simulink model "tb_pack_bms"  (R2026b)
model workspace (MAT data in the model file):
  TB.load_t = [0 10000000]
  TB.load_I = [0 0]
  TB.hv_t = [0 10000000]
  TB.hv_v = [0 0]
  TB.chg_t = [0 10000000]
  TB.chg_v = [0 0]
  TB.rst_t = [0 10000000]
  TB.rst_v = [0 0]
  TB.sd_t = [0 10000000]
  TB.sd_v = [0 0]
  TB.alive_freeze_t = 1000000000
  TB.dock_t = [0 10000000]
  TB.dock_v = [0 0]
  TB.shv_t = [0 10000000]
  TB.shv_v = [1 1]
  TB.sok_t = [0 10000000]
  TB.sok_v = [1 1]
  TB.T_amb = 298.15
  TB.G_solar = 0
  TB.chg_force = 0
  TB.chg_force_I = 100
  TB.flt_t = [0 10000000]
  TB.flt_v = [0 0]
  TB.fan_mode = 0
  TB.dec_fast = 1
  TB.dec_cmd = 1
  TB.V_gate = [30 35]
  TB.R_esr = 0.01
  TB.load_is_power = 0
  TB.stop_Vmin = 0
  TB.stop_SOCmin = -1
  TB.stop_SOCmax = 2
  TB.stop_on_done = 0
values from neighbouring files (symbols this model uses):
  P = local_temp(P, 318.15)    [pwr_case_def.m]    (also in pwr_case_run.m = C.pmod(P))
undefined symbols (not defined in the file or in its folder): Ts
libraries: simulink x15, nesl_utility x10, fl_lib x7, ee_lib x6, eeGeneralControl x4
settings Model: Creator=aomar  LastModifiedBy=aomar

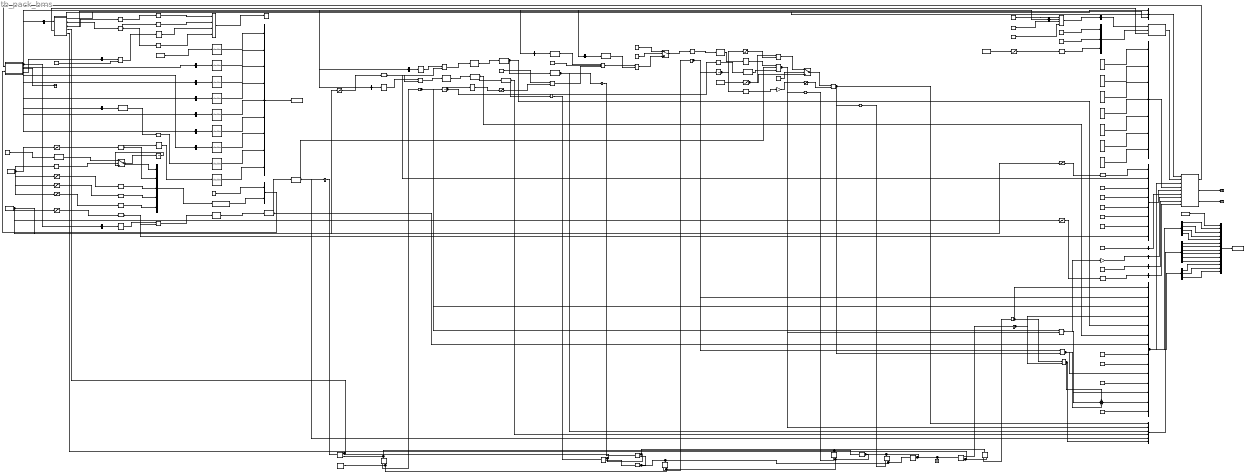
== system tb_pack_bms ==
  BMS : ModelReference  ModelNameDialog=Shaddad_BMS  SimulationMode=Normal  ModelReferenceVersion=1.1
  BMS_REQ_Pack : Subsystem  ReferencedSubsystem=bmsreq_can_pack
  Bal_log_sel : BusSelector  OutputSignals=Bal_Cmd
  Bal_sel : BusSelector  OutputSignals=Bal_Cmd
  Battery_Pack : Subsystem  Variant=on
  BmsReq_BC : BusCreator  Inputs=5  OutDataTypeStr=Bus: Bus_BmsReq  NonVirtualBus=on
      settings: InheritFromInputs=off
  C_bus : ee_lib/Passive/Capacitor  cap_option=ee.enum.passive.capacitor.capOption.const  c=P.power.pdu.C_bus_total_assumed F  Cvec=[1e-05, 1e-06] F  Vvec=[0, 10] V  CV_table_symmetry=ee.enum.passive.capacitor.tableSymmetry.yes  f_vec=[1, 10] kHz  DFext_vec=[.8, 1.2]  enable_C_tol=ee.enum.toleranceApplication.none  averaging_period=0 s  C_tol=5  tol_distribution=ee.enum.toleranceDistribution.uniform  nSigma=4  r=TB.R_esr Ohm  g=P.power.pdu.g_bleed 1/Ohm  enable_operating_limits=ee.enum.enable.no  operating_limit_action=ee.enum.passive.reportOpLim.warn  max_working_voltage_range=[-25, 25] V  power_rating=1 W  maxTemperature=85 degC  thermalEnable=false  thermalMass=1 J/K  i_specify=off  i_priority=None  i=0 A  i_nominal_specify=off  i_nominal_value=1  i_nominal_unit=A  v_specify=off  v_priority=None  v=0 V  v_nominal_specify=off  v_nominal_value=1  v_nominal_unit=V  vc_specify=on  vc_priority=High  vc=0 V  vc_nominal_specify=off  vc_nominal_value=1  vc_nominal_unit=V  T_specify=off  T_priority=None  T=298.15 K  T_nominal_specify=off  T_nominal_value=1  T_nominal_unit=K
  CanSlow_BC : BusCreator  Inputs=2  OutDataTypeStr=Bus: Bus_Can1_McuSlow  NonVirtualBus=on
      settings: InheritFromInputs=off
  Ch2_ok : Constant  Value=true  OutDataTypeStr=boolean  SampleTime=Ts.base
  Ch_ok : Constant  Value=true  OutDataTypeStr=boolean  SampleTime=Ts.base
  Charger : fl_lib/Electrical/Electrical Sources/Controlled Current Source
  Charger_BC : BusCreator  Inputs=1
  Charger_PS : nesl_utility/Simulink-PS Converter  PhysicalDomain=network_engine_domain  SubClassName=ps_input  LeftPortType=input  RightPortType=output  PseudoPeriodic=off  Frequencies=[]  NoiseDistribution=none  NoiseParameters=[]  Unit=A  AffineConversion=off  FilteringAndDerivatives=zero  SimscapeFilterOrder=1  InputFilterTimeConstant=0.001  UdotUserProvided=0
  Chg_RT : RateTransition  OutPortSampleTime=Ts.base
  Chg_en_dbl : DataTypeConversion  OutDataTypeStr=double  SaturateOnIntegerOverflow=off  RndMeth=Floor
  Chg_en_sel : BusSelector  OutputSignals=Charger_Enable
  Chg_force : Constant  Value=TB.chg_force  SampleTime=Ts.bms_fast
  Chg_force_I : Constant  Value=TB.chg_force_I  SampleTime=Ts.bms_fast
  Chg_force_sw : Switch  Criteria=u2 ~= 0  SaturateOnIntegerOverflow=off  InputSameDT=off
  Chg_lag : eeGeneralControl/Low-Pass Filter (Discrete or Continuous)  K=1  T=P.power.charger.tau  B=inf  A=-inf  init_option=Specify as parameter  x0=0  Ts=Ts.bms_fast
  Chg_slew : RateLimiter  RisingSlewLimit=P.power.charger.slew  FallingSlewLimit=-P.power.charger.slew  SampleTimeMode=inherited
  Clock_100ms : DigitalClock  SampleTime=Ts.env
  Clock_10ms : DigitalClock  SampleTime=Ts.bms_fast
  Clock_1ms : DigitalClock  SampleTime=Ts.base
  Clock_1ms_load : DigitalClock  SampleTime=Ts.base
  Clock_1ms_tab : DigitalClock  SampleTime=Ts.base
  Clock_50ms : DigitalClock  SampleTime=Ts.can_slow
  Dock_tab : Lookup_n-D  NumberOfTableDimensions=1  BreakpointsForDimension1=TB.dock_t  Table=TB.dock_v  InterpMethod=Flat  ExtrapMethod=Clip  InternalRulePriority=Speed  RndMeth=Simplest
  Dock_tab_100ms : Lookup_n-D  NumberOfTableDimensions=1  BreakpointsForDimension1=TB.dock_t  Table=TB.dock_v  InterpMethod=Flat  ExtrapMethod=Clip  InternalRulePriority=Speed  RndMeth=Simplest
  Dock_tab_100ms_b : simulink/Logic and Bit Operations/Compare To Zero  relop=~=  OutDataTypeStr=boolean
  Dock_tab_b : simulink/Logic and Bit Operations/Compare To Zero  relop=~=  OutDataTypeStr=boolean
  EStop_none : Constant  Value=false  OutDataTypeStr=boolean  SampleTime=Ts.base
  Env_BC : BusCreator  Inputs=3
  Env_ps_BC : BusCreator  Inputs=1
  Fan_BC : BusCreator  Inputs=1
  Fan_cmd_sel : BusSelector  OutputSignals=Fan_Cmd
  Fan_mode : Constant  Value=TB.fan_mode  SampleTime=Ts.bms_fast
  Fan_off : Constant  Value=single(0)  OutDataTypeStr=single  SampleTime=Ts.bms_fast
  Fan_on : Constant  Value=single(1)  OutDataTypeStr=single  SampleTime=Ts.bms_fast
  Fan_sel : MultiPortSwitch  DataPortOrder=Zero-based contiguous  zeroidx=on  SaturateOnIntegerOverflow=off  InputSameDT=off
  Fault_tab : Lookup_n-D  NumberOfTableDimensions=1  BreakpointsForDimension1=TB.flt_t  Table=TB.flt_v  InterpMethod=Flat  ExtrapMethod=Clip  InternalRulePriority=Speed  RndMeth=Simplest
  Fault_tab_b : simulink/Logic and Bit Operations/Compare To Zero  relop=~=  OutDataTypeStr=boolean
  Flt_BC : BusCreator  Inputs=1
  Fuse24_ok : Constant  Value=true  OutDataTypeStr=boolean  SampleTime=Ts.base
  FuseMain_ok : Constant  Value=true  OutDataTypeStr=boolean  SampleTime=Ts.base
  Fuse_ok : Constant  Value=true(6,1)  OutDataTypeStr=boolean  SampleTime=Ts.base
  GND : fl_lib/Electrical/Electrical Elements/Electrical Reference
  G_solar : Constant  Value=TB.G_solar  SampleTime=Ts.env
  HV_req_RT : RateTransition  OutPortSampleTime=Ts.bms_fast
  I_chg : Product  Inputs=3
  I_chg_en : Product
  I_chg_law : MinMax  Inputs=3
  I_chg_max : Constant  Value=P.power.charger.I_max  SampleTime=Ts.bms_fast
  I_from_P : Product  Inputs=*/
  I_load : Product
  I_pmax : Product  Inputs=*/
  I_req_dbl : DataTypeConversion  OutDataTypeStr=double  SaturateOnIntegerOverflow=off  RndMeth=Floor
  I_req_sel : BusSelector  OutputSignals=Charger_I_Req_A
  I_shunt : fl_lib/Electrical/Electrical Sensors/Current Sensor
  I_shunt_out : nesl_utility/PS-Simulink Converter  PhysicalDomain=network_engine_domain  SubClassName=ps_output  LeftPortType=input  RightPortType=output  PseudoPeriodic=off  Frequencies=[]  VectorFormat=inherit  Unit=inherit  AffineConversion=off
  Impl_BC : BusCreator  Inputs=1
  Impl_cmd_none : Constant  Value=P.ic.Bus_CanFrame8  OutDataTypeStr=Bus: Bus_CanFrame8  SampleTime=Ts.can_slow
  K1 : ee_lib/Switches & Breakers/Relays/SPST Relay  block_choices=ee.enum.controlport.ps  R_closed=P.power.pdu.K1.R_closed Ohm  G_open=P.power.pdu.K1.G_open 1/Ohm  Threshold=0.5  exposemeasurement=ee.enum.exposemeasurement.hidden  V_rated=5 V  V_energize=75  V_deenergize=25  l_winding=0.08 H  r_winding=12.5 Ohm  g_winding=1e-9 1/Ohm  T_brk_C_S=0 s  T_mak_C_S=0 s  fault_types=ee.enum.relays.faultTypes.winding
  K1_Cmd_sel : BusSelector  OutputSignals=K1_Cmd
  K1_aux : DataTypeConversion  OutDataTypeStr=boolean  SaturateOnIntegerOverflow=off  RndMeth=Floor
  K1_aux_dbl : DataTypeConversion  OutDataTypeStr=double  SaturateOnIntegerOverflow=off  RndMeth=Floor
  K1_cmd_RT : RateTransition  OutPortSampleTime=Ts.base
  K1_coil : Logic  AllPortsSameDT=off  OutDataTypeStr=boolean
  K1_coil_PS : nesl_utility/Simulink-PS Converter  PhysicalDomain=network_engine_domain  SubClassName=ps_input  LeftPortType=input  RightPortType=output  PseudoPeriodic=off  Frequencies=[]  NoiseDistribution=none  NoiseParameters=[]  Unit=1  AffineConversion=off  FilteringAndDerivatives=zero  SimscapeFilterOrder=1  InputFilterTimeConstant=0.001  UdotUserProvided=0
  K1_delay : eeGeneralControl/On-Off Delay  LabelModeActiveChoice=Discrete  Td_on=P.power.pdu.K1.t_on  Td_off=P.power.pdu.K1.t_off  IC=0  Ts=Ts.base
      settings: LibrarySourceBlock=ee_sl_lib/General Control/On-Off Delay
  K2 : ee_lib/Switches & Breakers/Relays/SPST Relay  block_choices=ee.enum.controlport.ps  R_closed=P.power.pdu.K2.R_closed Ohm  G_open=P.power.pdu.K2.G_open 1/Ohm  Threshold=0.5  exposemeasurement=ee.enum.exposemeasurement.hidden  V_rated=5 V  V_energize=75  V_deenergize=25  l_winding=0.08 H  r_winding=12.5 Ohm  g_winding=1e-9 1/Ohm  T_brk_C_S=0 s  T_mak_C_S=0 s  fault_types=ee.enum.relays.faultTypes.winding
  K2_Cmd_sel : BusSelector  OutputSignals=K2_Cmd
  K2_aux : DataTypeConversion  OutDataTypeStr=boolean  SaturateOnIntegerOverflow=off  RndMeth=Floor
  K2_aux_dbl : DataTypeConversion  OutDataTypeStr=double  SaturateOnIntegerOverflow=off  RndMeth=Floor
  K2_cmd_RT : RateTransition  OutPortSampleTime=Ts.base
  K2_coil : Logic  AllPortsSameDT=off  OutDataTypeStr=boolean
  K2_coil_PS : nesl_utility/Simulink-PS Converter  PhysicalDomain=network_engine_domain  SubClassName=ps_input  LeftPortType=input  RightPortType=output  PseudoPeriodic=off  Frequencies=[]  NoiseDistribution=none  NoiseParameters=[]  Unit=1  AffineConversion=off  FilteringAndDerivatives=zero  SimscapeFilterOrder=1  InputFilterTimeConstant=0.001  UdotUserProvided=0
  K2_delay : eeGeneralControl/On-Off Delay  LabelModeActiveChoice=Discrete  Td_on=P.power.pdu.K2.t_on  Td_off=P.power.pdu.K2.t_off  IC=0  Ts=Ts.base
      settings: LibrarySourceBlock=ee_sl_lib/General Control/On-Off Delay
  K3_none : Constant  Value=false  OutDataTypeStr=boolean  SampleTime=Ts.base
  K4 : ee_lib/Switches & Breakers/Relays/SPST Relay  block_choices=ee.enum.controlport.ps  R_closed=P.power.pdu.K4.R_closed Ohm  G_open=P.power.pdu.K4.G_open 1/Ohm  Threshold=0.5  exposemeasurement=ee.enum.exposemeasurement.hidden  V_rated=5 V  V_energize=75  V_deenergize=25  l_winding=0.08 H  r_winding=12.5 Ohm  g_winding=1e-9 1/Ohm  T_brk_C_S=0 s  T_mak_C_S=0 s  fault_types=ee.enum.relays.faultTypes.winding
  K4_Cmd_sel : BusSelector  OutputSignals=K4_Cmd
  K4_aux : DataTypeConversion  OutDataTypeStr=boolean  SaturateOnIntegerOverflow=off  RndMeth=Floor
  K4_aux_dbl : DataTypeConversion  OutDataTypeStr=double  SaturateOnIntegerOverflow=off  RndMeth=Floor
  K4_cmd_RT : RateTransition  OutPortSampleTime=Ts.base
  K4_coil : Logic  AllPortsSameDT=off  OutDataTypeStr=boolean
  K4_coil_PS : nesl_utility/Simulink-PS Converter  PhysicalDomain=network_engine_domain  SubClassName=ps_input  LeftPortType=input  RightPortType=output  PseudoPeriodic=off  Frequencies=[]  NoiseDistribution=none  NoiseParameters=[]  Unit=1  AffineConversion=off  FilteringAndDerivatives=zero  SimscapeFilterOrder=1  InputFilterTimeConstant=0.001  UdotUserProvided=0
  K4_delay : eeGeneralControl/On-Off Delay  LabelModeActiveChoice=Discrete  Td_on=P.power.pdu.K4.t_on  Td_off=P.power.pdu.K4.t_off  IC=0  Ts=Ts.base
      settings: LibrarySourceBlock=ee_sl_lib/General Control/On-Off Delay
  Key_on : Constant  Value=true  OutDataTypeStr=boolean  SampleTime=Ts.base
  Latched_none : Constant  Value=false  OutDataTypeStr=boolean  SampleTime=Ts.base
  Load : fl_lib/Electrical/Electrical Sources/Controlled Current Source
  Load_PS : nesl_utility/Simulink-PS Converter  PhysicalDomain=network_engine_domain  SubClassName=ps_input  LeftPortType=input  RightPortType=output  PseudoPeriodic=off  Frequencies=[]  NoiseDistribution=none  NoiseParameters=[]  Unit=A  AffineConversion=off  FilteringAndDerivatives=zero  SimscapeFilterOrder=1  InputFilterTimeConstant=0.001  UdotUserProvided=0
  Load_is_power : Constant  Value=TB.load_is_power  SampleTime=Ts.base
  Load_mode : Switch  Criteria=u2 ~= 0  SaturateOnIntegerOverflow=off  InputSameDT=off
  Load_tab : Lookup_n-D  NumberOfTableDimensions=1  BreakpointsForDimension1=TB.load_t  Table=TB.load_I  InterpMethod=Flat  ExtrapMethod=Clip  InternalRulePriority=Speed  RndMeth=Simplest
  Log_Charger_Enable_sel : BusSelector  OutputSignals=Charger_Enable
  Log_Charger_I_Req_A_sel : BusSelector  OutputSignals=Charger_I_Req_A
  Log_Fan_Cmd_sel : BusSelector  OutputSignals=Fan_Cmd
  Log_K1_Cmd_sel : BusSelector  OutputSignals=K1_Cmd
  Log_K2_Cmd_sel : BusSelector  OutputSignals=K2_Cmd
  Log_K4_Cmd_sel : BusSelector  OutputSignals=K4_Cmd
  Log_meas_sel : BusSelector  OutputSignals=V_pack,V_bus,V_dock,I_pack
  Log_pwr_sel : BusSelector  OutputSignals=P_trac_L,P_chg_bus,P_pdu_loss
  Log_stub_BC : BusCreator  Inputs=6
  Log_stub_sel : BusSelector  OutputSignals=I_load,I_chg,K1_closed_dbl,K2_closed_dbl,K4_closed_dbl,P_pack
  Lv_BC : BusCreator  Inputs=7
  MCU_Charge_Enable_Req : Lookup_n-D  NumberOfTableDimensions=1  BreakpointsForDimension1=TB.chg_t  Table=TB.chg_v  InterpMethod=Flat  ExtrapMethod=Clip  InternalRulePriority=Speed  RndMeth=Simplest
  MCU_Charge_Enable_Req_b : simulink/Logic and Bit Operations/Compare To Zero  relop=~=  OutDataTypeStr=boolean
  MCU_Fault_Reset_Req : Lookup_n-D  NumberOfTableDimensions=1  BreakpointsForDimension1=TB.rst_t  Table=TB.rst_v  InterpMethod=Flat  ExtrapMethod=Clip  InternalRulePriority=Speed  RndMeth=Simplest
  MCU_Fault_Reset_Req_b : simulink/Logic and Bit Operations/Compare To Zero  relop=~=  OutDataTypeStr=boolean
  MCU_HV_Enable_Req : Lookup_n-D  NumberOfTableDimensions=1  BreakpointsForDimension1=TB.hv_t  Table=TB.hv_v  InterpMethod=Flat  ExtrapMethod=Clip  InternalRulePriority=Speed  RndMeth=Simplest
  MCU_HV_Enable_Req_b : simulink/Logic and Bit Operations/Compare To Zero  relop=~=  OutDataTypeStr=boolean
  MCU_Shutdown_Req : Lookup_n-D  NumberOfTableDimensions=1  BreakpointsForDimension1=TB.sd_t  Table=TB.sd_v  InterpMethod=Flat  ExtrapMethod=Clip  InternalRulePriority=Speed  RndMeth=Simplest
  MCU_Shutdown_Req_b : simulink/Logic and Bit Operations/Compare To Zero  relop=~=  OutDataTypeStr=boolean
  MCU_alive : simulink/Sources/Counter Free-Running  NumBits=8  tsamp=Ts.can_slow
  MCU_alive_hold : UnitDelay  InitialCondition=uint8(0)  SampleTime=Ts.can_slow
  MCU_alive_run : simulink/Logic and Bit Operations/Compare To Constant  relop=<  const=TB.alive_freeze_t  OutDataTypeStr=boolean
  MCU_alive_sw : Switch  Criteria=u2 ~= 0  SaturateOnIntegerOverflow=off  InputSameDT=off
  MCU_alive_u8 : DataTypeConversion  OutDataTypeStr=uint8  SaturateOnIntegerOverflow=off  RndMeth=Floor
  OVP_ok : simulink/Logic and Bit Operations/Compare To Constant  relop=<  const=P.power.charger.V_ovp  OutDataTypeStr=boolean
  OVP_ok_dbl : DataTypeConversion  OutDataTypeStr=double  SaturateOnIntegerOverflow=off  RndMeth=Floor
  P_chg_bus : Product
  P_chg_max : Constant  Value=P.power.charger.P_max  SampleTime=Ts.bms_fast
  P_grid : Gain  Gain=1/P.power.charger.eta
  P_pack : Product
  P_pdu_loss : Sum  Inputs=++-
  P_trac : Product
  Pack_BC : BusCreator  Inputs=3
  Pack_Thermal : Subsystem  ReferencedSubsystem=Pack_Thermal
  Pdu_BC : BusCreator  Inputs=14
  Power_Sensors : Subsystem  ReferencedSubsystem=Power_Sensors
  R_dock_bleed : ee_lib/Passive/Resistor  R=P.power.charger.R_bleed Ohm  enable_R_tol=ee.enum.toleranceApplication.none  R_tol=5  tol_distribution=ee.enum.toleranceDistribution.uniform  nSigma=4  enable_operating_limits=ee.enum.enable.no  operating_limit_action=ee.enum.passive.reportOpLim.warn  power_rating=1 W  max_working_voltage=100 V  noise_mode=ee.enum.sources.noise.Disabled  Tdevice=25 degC  sample_time=1e-3 s  repeatability=ee.enum.ic.repeatability.notRepeatable  user_seed=0  auto_seed=2562091618  power_derating_T1=70 degC  power_derating_T2=155 degC  operating_temperature_range_vec=[-50, 150] degC  alpha=3.93e-3 1/K  Tmeas=25 degC  thermal_mass=100 J/K  temperature_specify=off  temperature_priority=High  temperature=298.15 K  temperature_nominal_specify=off  temperature_nominal_value=1  temperature_nominal_unit=K
  R_pre : ee_lib/Passive/Resistor  R=P.power.pdu.R_pre Ohm  enable_R_tol=ee.enum.toleranceApplication.none  R_tol=5  tol_distribution=ee.enum.toleranceDistribution.uniform  nSigma=4  enable_operating_limits=ee.enum.enable.no  operating_limit_action=ee.enum.passive.reportOpLim.warn  power_rating=1 W  max_working_voltage=100 V  noise_mode=ee.enum.sources.noise.Disabled  Tdevice=25 degC  sample_time=1e-3 s  repeatability=ee.enum.ic.repeatability.notRepeatable  user_seed=0  auto_seed=4166091829  power_derating_T1=70 degC  power_derating_T2=155 degC  operating_temperature_range_vec=[-50, 150] degC  alpha=3.93e-3 1/K  Tmeas=25 degC  thermal_mass=100 J/K  temperature_specify=off  temperature_priority=High  temperature=298.15 K  temperature_nominal_specify=off  temperature_nominal_value=1  temperature_nominal_unit=K
  Rails : Constant  Value=[24; 2; 24; 12; 4; 5; 3.3]  SampleTime=Ts.base
  Rails_ok : Constant  Value=true(4,1)  OutDataTypeStr=boolean  SampleTime=Ts.base
  SOC_min_true : MinMax
  Safety_BC : BusCreator  Inputs=8
  Safety_HV_OK_tab : Lookup_n-D  NumberOfTableDimensions=1  BreakpointsForDimension1=TB.shv_t  Table=TB.shv_v  InterpMethod=Flat  ExtrapMethod=Clip  InternalRulePriority=Speed  RndMeth=Simplest
  Safety_HV_OK_tab_b : simulink/Logic and Bit Operations/Compare To Zero  relop=~=  OutDataTypeStr=boolean
  Safety_OK_tab : Lookup_n-D  NumberOfTableDimensions=1  BreakpointsForDimension1=TB.sok_t  Table=TB.sok_v  InterpMethod=Flat  ExtrapMethod=Clip  InternalRulePriority=Speed  RndMeth=Simplest
  Safety_OK_tab_b : simulink/Logic and Bit Operations/Compare To Zero  relop=~=  OutDataTypeStr=boolean
  Solver : nesl_utility/Solver Configuration  PhysicalDomain=network_engine_domain  SubClassName=solver  LeftPortType=input  RightPortType=generic  Tones=[]  Harmonics=[]  SimulateNoise=off  Profile=off  UseLocalSampling=off  EnableSwitchedLinearOptims=on  FrequencyDomain=off  UseCCode=off  RelTol=0.001  AbsTol=0.001  MinStep=1e-09  ToWorkspace=off  RevertToSquareIcSolve=off  NumHomotopyIterations=100  PhasorMode=off  PhasorModeNumHarmonics=1  ConsistencySolver=NEWTON_XTOL_AFTER_FTOL  CanonicalOrdering=CANONICAL  OptimizeIntermediates=OPTIMIZED  MulticoreSolverChoice=BACKWARD_EULER  IndexReductionMethod=DerivativeReplacement  DoDC=off  ResidualTolerance=1e-09  ConsistencyTolSource=GLOBAL  ConsistencyAbsTol=0.001  ConsistencyRelTol=0.001  ConsistencyTolFactor=0.001  UseLocalSolver=on  LocalSolverChoice=NE_BACKWARD_EULER_ADVANCER  ResolveIndetEquations=on  FunctionEvalNumThread=1  LocalSolverSampleTime=P.sim.ssc.Ts  DoFixedCost=on  MaxNonlinIter=P.power.tb.MaxNonlinIter  MaxModeIter=P.power.tb.MaxModeIter  ComputeImpulses=off  ImpulseIterations=2  LinearAlgebra=auto  LinearAlgebraNumThread=0  EquationFormulation=NE_TIME_EF  DelaysMemoryBudget=1024  AutomaticFiltering=on  FilteringTimeConstant=0.001  PartitionStorageMethod=AS_NEEDED  PartitionMemoryBudget=1024  PartitionMethod=BALANCED  MultibodyUseLocalSolver=off  MultibodyLocalSolverChoice=ODE1  MultibodyLocalSolverSampleTime=0.001
  Stop : Stop
  Stop_SOC : simulink/Logic and Bit Operations/Compare To Constant  relop=<  const=TB.stop_SOCmin  OutDataTypeStr=boolean
  Stop_SOCmax : simulink/Logic and Bit Operations/Compare To Constant  relop=>  const=TB.stop_SOCmax  OutDataTypeStr=boolean
  Stop_V : simulink/Logic and Bit Operations/Compare To Constant  relop=<  const=TB.stop_Vmin  OutDataTypeStr=boolean
  Stop_any : Logic  Operator=OR  Inputs=4  AllPortsSameDT=off  OutDataTypeStr=boolean
  Stop_done : Logic  AllPortsSameDT=off  OutDataTypeStr=boolean
  Stop_done_RT : RateTransition  OutPortSampleTime=Ts.base
  Stop_on_done : Constant  Value=TB.stop_on_done  OutDataTypeStr=boolean  SampleTime=Ts.hk
  T_amb : Constant  Value=TB.T_amb  SampleTime=Ts.env
  T_amb_ps : Constant  Value=TB.T_amb  SampleTime=Ts.env
  Telem_sel : BusSelector  OutputSignals=Charge_Complete
  V_bus_d : UnitDelay  SampleTime=Ts.base
  V_bus_min : Saturate  UpperLimit=inf  LowerLimit=30
  V_bus_sens : fl_lib/Electrical/Electrical Sensors/Voltage Sensor
  V_bus_sens_out : nesl_utility/PS-Simulink Converter  PhysicalDomain=network_engine_domain  SubClassName=ps_output  LeftPortType=input  RightPortType=output  PseudoPeriodic=off  Frequencies=[]  VectorFormat=inherit  Unit=inherit  AffineConversion=off
  V_dock_RT : RateTransition  OutPortSampleTime=Ts.bms_fast
  V_dock_d : UnitDelay  SampleTime=Ts.base
  V_dock_min : Saturate  UpperLimit=inf  LowerLimit=1
  V_dock_sens : fl_lib/Electrical/Electrical Sensors/Voltage Sensor
  V_dock_sens_out : nesl_utility/PS-Simulink Converter  PhysicalDomain=network_engine_domain  SubClassName=ps_output  LeftPortType=input  RightPortType=output  PseudoPeriodic=off  Frequencies=[]  VectorFormat=inherit  Unit=inherit  AffineConversion=off
  V_gate : Saturate  UpperLimit=1  LowerLimit=0
  V_gate_k : Gain  Gain=1/(TB.V_gate(2) - TB.V_gate(1))
  V_gate_off : Bias  Bias=-TB.V_gate(1)  SaturateOnIntegerOverflow=off
  V_pack_sens : fl_lib/Electrical/Electrical Sensors/Voltage Sensor
  V_pack_sens_out : nesl_utility/PS-Simulink Converter  PhysicalDomain=network_engine_domain  SubClassName=ps_output  LeftPortType=input  RightPortType=output  PseudoPeriodic=off  Frequencies=[]  VectorFormat=inherit  Unit=inherit  AffineConversion=off
  Vcell_min_true : MinMax
  Zero_P_bms : Constant  Value=0  SampleTime=Ts.base
  Zero_P_dcdc_loss : Constant  Value=0  SampleTime=Ts.base
  Zero_P_impl : Constant  Value=0  SampleTime=Ts.base
  Zero_P_k3_loss : Constant  Value=0  SampleTime=Ts.base
  Zero_P_lv : Constant  Value=0  SampleTime=Ts.base
  Zero_P_trac_R : Constant  Value=0  SampleTime=Ts.base
  can_tx_term : Terminator
  lc_dbl{1..9} (9 alike) : DataTypeConversion  OutDataTypeStr=double  SaturateOnIntegerOverflow=off  RndMeth=Floor
  log_cmd : ToWorkspace  VariableName=log_cmd  SampleTime=-1
      settings: Decimation=TB.dec_cmd
  log_cmd_mux : Mux  Inputs=9
  log_fast : ToWorkspace  VariableName=log_fast  SampleTime=-1
      settings: Decimation=TB.dec_fast
  log_fast_mux : Mux  Inputs=14
  n_bal_dbl : DataTypeConversion  OutDataTypeStr=double  SaturateOnIntegerOverflow=off  RndMeth=Floor
  n_bal_sum : Sum  Inputs=+
  status_term : Terminator
  truth_term : Terminator
  wires:
  MCU_alive/1 -> MCU_alive_u8/1  "alive_count"
  Clock_1ms_tab/1 -> Safety_HV_OK_tab/1, Safety_OK_tab/1, Fault_tab/1, Dock_tab/1  "t_1ms_tab"
  Clock_50ms/1 -> MCU_HV_Enable_Req/1, MCU_Shutdown_Req/1, MCU_Fault_Reset_Req/1, MCU_alive_run/1, MCU_Charge_Enable_Req/1  "t_50ms"
  BMS/1 -> K4_Cmd_sel/1, Log_Fan_Cmd_sel/1, Log_Charger_I_Req_A_sel/1, Log_Charger_Enable_sel/1, Fan_cmd_sel/1, Bal_sel/1, Bal_log_sel/1, Log_K4_Cmd_sel/1, K2_Cmd_sel/1, Log_K2_Cmd_sel/1, I_req_sel/1, Chg_en_sel/1, K1_Cmd_sel/1, Log_K1_Cmd_sel/1  "bms_cmd"
  BMS/2 -> can_tx_term/1  "can_tx"
  BMS/3 -> Telem_sel/1  "telem"
  Bal_sel/1 -> Battery_Pack/1(Bal_Cmd)  "<Bal_Cmd>"
  Stop_on_done/1 -> Stop_done/2  "stop_on_done"
  MCU_alive_run/1 -> MCU_alive_sw/2  "alive_running"
  MCU_HV_Enable_Req/1 -> MCU_HV_Enable_Req_b/1  "HV_Enable_Req_tab"
  MCU_Charge_Enable_Req/1 -> MCU_Charge_Enable_Req_b/1  "Charge_Enable_Req_tab"
  MCU_Fault_Reset_Req/1 -> MCU_Fault_Reset_Req_b/1  "Fault_Reset_Req_tab"
  MCU_Shutdown_Req/1 -> MCU_Shutdown_Req_b/1  "Shutdown_Req_tab"
  Dock_tab/1 -> Dock_tab_b/1  "dock_present_tab"
  MCU_alive_u8/1 -> MCU_alive_sw/1  "alive_count_u8"
  Battery_Pack/1(T_cell_true) -> Pack_BC/1  "T_cell_true"
  Telem_sel/1 -> Stop_done/1  "<Charge_Complete>"
  Bal_log_sel/1 -> n_bal_dbl/1  "<Bal_Cmd>"
  K4_Cmd_sel/1 -> K4_cmd_RT/1  "<K4_Cmd>"
  Vcell_min_true/1 -> Stop_V/1  "V_cell_min"
  SOC_min_true/1 -> Stop_SOCmax/1, Stop_SOC/1  "SOC_min"
  Stop_done/1 -> Stop_done_RT/1  "stop_done"
  MCU_HV_Enable_Req_b/1 -> BmsReq_BC/2, HV_req_RT/1  "HV_Enable_Req"
  MCU_Charge_Enable_Req_b/1 -> BmsReq_BC/3  "Charge_Enable_Req"
  MCU_Fault_Reset_Req_b/1 -> BmsReq_BC/4  "Fault_Reset_Req"
  MCU_Shutdown_Req_b/1 -> BmsReq_BC/5  "Shutdown_Req"
  Dock_tab_b/1 -> Safety_BC/8, K4_coil/2  "dock_present"
  K4_cmd_RT/1 -> K4_coil/1  "K4_Cmd_1ms"
  MCU_alive_sw/1 -> MCU_alive_hold/1, BmsReq_BC/1  "AliveCounter"
  n_bal_dbl/1 -> n_bal_sum/1  "Bal_Cmd_dbl"
  BmsReq_BC/1 -> BMS_REQ_Pack/1  "bms_req"
  Stop_V/1 -> Stop_any/1  "stop_V"
  Stop_SOC/1 -> Stop_any/2  "stop_SOC"
  Stop_SOCmax/1 -> Stop_any/4  "stop_SOCmax"
  n_bal_sum/1 -> lc_dbl8/1  "n_Bal"
  K4_coil/1 -> K4_delay/1  "K4_coil"
  MCU_alive_hold/1 -> MCU_alive_sw/3  "alive_held"
  Stop_done_RT/1 -> Stop_any/3  "stop_done_1ms"
  HV_req_RT/1 -> lc_dbl9/1  "HV_Enable_Req_10ms"
  Clock_10ms/1 -> lc_dbl1/1  "t_10ms"
  Log_K1_Cmd_sel/1 -> lc_dbl2/1  "<K1_Cmd>"
  Log_K2_Cmd_sel/1 -> lc_dbl3/1  "<K2_Cmd>"
  Log_K4_Cmd_sel/1 -> lc_dbl4/1  "<K4_Cmd>"
  Log_Charger_Enable_sel/1 -> lc_dbl5/1  "<Charger_Enable>"
  Log_Charger_I_Req_A_sel/1 -> lc_dbl6/1  "<Charger_I_Req_A>"
  Log_Fan_Cmd_sel/1 -> lc_dbl7/1  "<Fan_Cmd>"
  Stop_any/1 -> Stop/1  "stop_run"
  Impl_cmd_none/1 -> CanSlow_BC/1  "impl_cmd"
  K4_delay/1 -> K4_aux/1  "K4_contact"
  lc_dbl1/1 -> log_cmd_mux/1  "t_dbl"
  lc_dbl2/1 -> log_cmd_mux/2  "K1_Cmd_dbl"
  lc_dbl3/1 -> log_cmd_mux/3  "K2_Cmd_dbl"
  lc_dbl4/1 -> log_cmd_mux/4  "K4_Cmd_dbl"
  lc_dbl5/1 -> log_cmd_mux/5  "Charger_Enable_dbl"
  lc_dbl6/1 -> log_cmd_mux/6  "I_req_dbl"
  lc_dbl7/1 -> log_cmd_mux/7  "Fan_Cmd_dbl"
  lc_dbl8/1 -> log_cmd_mux/8  "n_Bal_dbl"
  lc_dbl9/1 -> log_cmd_mux/9  "HV_Enable_Req_MCU_dbl"
  BMS_REQ_Pack/1 -> CanSlow_BC/2  "bms_req"
  log_cmd_mux/1 -> log_cmd/1  "log_cmd"
  CanSlow_BC/1 -> BMS/2  "can_rx"
  K4_aux/1 -> Pdu_BC/7, K4_aux_dbl/1  "K4_closed"
  K4_aux_dbl/1 -> Log_stub_BC/5, I_chg/2, K4_coil_PS/1  "K4_closed_dbl"
  Safety_HV_OK_tab/1 -> Safety_HV_OK_tab_b/1  "Safety_HV_OK_tab"
  K2_Cmd_sel/1 -> K2_cmd_RT/1  "<K2_Cmd>"
  Safety_HV_OK_tab_b/1 -> Safety_BC/2, K2_coil/2, K1_coil/2  "Safety_HV_OK"
  K2_cmd_RT/1 -> K2_coil/1  "K2_Cmd_1ms"
  K1_Cmd_sel/1 -> K1_cmd_RT/1  "<K1_Cmd>"
  V_dock_sens_out/1 -> P_chg_bus/1, Pdu_BC/3, V_dock_d/1  "V_dock"
  K2_coil/1 -> K2_delay/1  "K2_coil"
  K1_cmd_RT/1 -> K1_coil/1  "K1_Cmd_1ms"
  K1_coil/1 -> K1_delay/1  "K1_coil"
  V_dock_d/1 -> OVP_ok/1, V_dock_RT/1  "V_dock_d"
  K2_delay/1 -> K2_aux/1  "K2_contact"
  V_dock_RT/1 -> V_dock_min/1  "V_dock_10ms"
  K1_delay/1 -> K1_aux/1  "K1_contact"
  K2_aux/1 -> Pdu_BC/6, K2_aux_dbl/1  "K2_closed"
  P_chg_max/1 -> I_pmax/1  "P_chg_max"
  V_dock_min/1 -> I_pmax/2  "V_dock_min"
  K1_aux/1 -> Pdu_BC/5, K1_aux_dbl/1  "K1_closed"
  K2_aux_dbl/1 -> Log_stub_BC/4, K2_coil_PS/1  "K2_closed_dbl"
  I_req_sel/1 -> I_req_dbl/1  "<Charger_I_Req_A>"
  I_chg_max/1 -> I_chg_law/2  "I_chg_max"
  I_pmax/1 -> I_chg_law/3  "I_pmax"
  I_req_dbl/1 -> I_chg_law/1  "I_req"
  K1_aux_dbl/1 -> Log_stub_BC/3, K1_coil_PS/1  "K1_closed_dbl"
  Chg_en_sel/1 -> Chg_en_dbl/1  "<Charger_Enable>"
  I_chg_law/1 -> I_chg_en/1  "I_chg_law"
  Chg_en_dbl/1 -> I_chg_en/2  "charger_enable"
  Chg_force_I/1 -> Chg_force_sw/1  "chg_force_I"
  Chg_force/1 -> Chg_force_sw/2  "chg_force"
  I_chg_en/1 -> Chg_force_sw/3  "I_chg_cmd"
  Chg_force_sw/1 -> Chg_slew/1  "I_chg_target"
  V_bus_sens_out/1 -> P_trac/1, Pdu_BC/2, V_bus_d/1  "V_bus"
  Chg_slew/1 -> Chg_lag/1  "I_chg_slewed"
  OVP_ok/1 -> OVP_ok_dbl/1  "ovp_ok"
  V_bus_d/1 -> V_bus_min/1, V_gate_off/1  "V_bus_d"
  Clock_1ms_load/1 -> Load_tab/1  "t_1ms_load"
  Chg_lag/1 -> Chg_RT/1  "I_chg_set"
  V_bus_min/1 -> I_from_P/2  "V_bus_d_min"
  Chg_RT/1 -> I_chg/1  "I_chg_set_1ms"
  Load_tab/1 -> I_from_P/1, Load_mode/3  "load_tab"
  V_gate_off/1 -> V_gate_k/1  "V_gate_dV"
  OVP_ok_dbl/1 -> I_chg/3  "ovp_ok_dbl"
  I_from_P/1 -> Load_mode/1  "I_from_P"
  I_chg/1 -> Log_stub_BC/2, P_chg_bus/2, Charger_PS/1  "I_chg"
  Load_is_power/1 -> Load_mode/2  "load_is_power"
  V_gate_k/1 -> V_gate/1  "V_gate_raw"
  V_gate/1 -> I_load/2  "V_gate"
  Load_mode/1 -> I_load/1  "I_load_req"
  I_load/1 -> Log_stub_BC/1, P_trac/2, Load_PS/1  "I_load"
  Clock_100ms/1 -> Dock_tab_100ms/1  "t_100ms"
  V_pack_sens_out/1 -> P_pack/1, Pdu_BC/1  "V_pack"
  I_shunt_out/1 -> P_pack/2, Pdu_BC/4  "I_pack"
  Fan_mode/1 -> Fan_sel/1  "fan_mode"
  Fan_off/1 -> Fan_sel/3  "fan_off"
  Fan_on/1 -> Fan_sel/4  "fan_on"
  Dock_tab_100ms/1 -> Dock_tab_100ms_b/1  "dock_contact_tab"
  Fan_cmd_sel/1 -> Fan_sel/2  "<Fan_Cmd>"
  T_amb/1 -> Env_BC/1  "T_amb"
  G_solar/1 -> Env_BC/2  "G_solar"
  P_chg_bus/1 -> P_grid/1, P_pdu_loss/2, Pdu_BC/12  "P_chg_bus"
  Fan_sel/1 -> Fan_BC/1  "Fan_Cmd"
  Dock_tab_100ms_b/1 -> Env_BC/3  "dock_contact"
  Safety_OK_tab/1 -> Safety_OK_tab_b/1  "Safety_OK_tab"
  Fault_tab/1 -> Fault_tab_b/1  "bms_fault_tab"
  P_trac/1 -> P_pdu_loss/3, Pdu_BC/10  "P_trac_L"
  P_pack/1 -> Log_stub_BC/6, P_pdu_loss/1  "P_pack"
  Fan_BC/1 -> Pack_Thermal/1  "fan_cmd"
  Env_BC/1 -> Pack_Thermal/2  "env"
  P_pdu_loss/1 -> Pdu_BC/13  "P_pdu_loss"
  Rails/1 -> Lv_BC/1  "rails"
  Rails_ok/1 -> Lv_BC/2  "rail_ok"
  K3_none/1 -> Lv_BC/3  "K3_closed"
  Fuse24_ok/1 -> Lv_BC/4  "fuse24_ok"
  Zero_P_lv/1 -> Lv_BC/5  "P_lv"
  Zero_P_dcdc_loss/1 -> Lv_BC/6  "P_dcdc_loss"
  Zero_P_k3_loss/1 -> Lv_BC/7  "P_k3_loss"
  EStop_none/1 -> Safety_BC/3  "EStop_Any"
  Ch_ok/1 -> Safety_BC/4  "EStop_Ch1_OK"
  Ch2_ok/1 -> Safety_BC/5  "EStop_Ch2_OK"
  Latched_none/1 -> Safety_BC/6  "Safety_Latched_Off"
  Key_on/1 -> Safety_BC/7  "key_on"
  Zero_P_impl/1 -> Impl_BC/1  "P_impl"
  P_grid/1 -> Charger_BC/1  "P_grid"
  T_amb_ps/1 -> Env_ps_BC/1  "T_amb"
  Fuse_ok/1 -> Pdu_BC/8  "fuse_ok"
  FuseMain_ok/1 -> Pdu_BC/9  "F_MAIN_ok"
  Zero_P_trac_R/1 -> Pdu_BC/11  "P_trac_R"
  Zero_P_bms/1 -> Pdu_BC/14  "P_bms"
  Safety_OK_tab_b/1 -> Safety_BC/1  "Safety_OK"
  Fault_tab_b/1 -> Flt_BC/1  "bms_fault"
  Pack_BC/1 -> Power_Sensors/1  "pack"
  Lv_BC/1 -> Power_Sensors/4  "lv"
  Safety_BC/1 -> Power_Sensors/5  "safety"
  Impl_BC/1 -> Power_Sensors/6  "impl"
  Charger_BC/1 -> Power_Sensors/7  "charger"
  Env_ps_BC/1 -> Power_Sensors/8  "env"
  Flt_BC/1 -> Power_Sensors/9  "flt"
  Pdu_BC/1 -> Power_Sensors/3, Log_meas_sel/1, Log_pwr_sel/1  "pdu"
  Log_stub_BC/1 -> Log_stub_sel/1  "log_stub"
  Pack_Thermal/1 -> Power_Sensors/2  "thermal"
  Log_meas_sel/1 -> log_fast_mux/2  "<V_pack>"
  Log_meas_sel/2 -> log_fast_mux/3  "<V_bus>"
  Log_meas_sel/3 -> log_fast_mux/4  "<V_dock>"
  Log_meas_sel/4 -> log_fast_mux/5  "<I_pack>"
  Log_stub_sel/1 -> log_fast_mux/6  "<I_load>"
  Log_stub_sel/2 -> log_fast_mux/7  "<I_chg>"
  Log_stub_sel/3 -> log_fast_mux/8  "<K1_closed_dbl>"
  Log_stub_sel/4 -> log_fast_mux/9  "<K2_closed_dbl>"
  Log_stub_sel/5 -> log_fast_mux/10  "<K4_closed_dbl>"
  Log_stub_sel/6 -> log_fast_mux/11  "<P_pack>"
  Log_pwr_sel/1 -> log_fast_mux/12  "<P_trac_L>"
  Log_pwr_sel/2 -> log_fast_mux/13  "<P_chg_bus>"
  Log_pwr_sel/3 -> log_fast_mux/14  "<P_pdu_loss>"
  Clock_1ms/1 -> log_fast_mux/1  "t_1ms"
  Power_Sensors/1 -> BMS/1  "bms_meas"
  Power_Sensors/2 -> status_term/1  "power_status"
  Power_Sensors/3 -> truth_term/1  "power_truth"
  log_fast_mux/1 -> log_fast/1  "log_fast"
  Battery_Pack/2(SOC_true) -> SOC_min_true/1, Pack_BC/2  "SOC_true"
  Battery_Pack/3(V_cell_true) -> Pack_BC/3, Vcell_min_true/1  "V_cell_true"
  connections:
  Battery_Pack/LConn1 -- Pack_Thermal/LConn1
  K4/RConn1 -- Battery_Pack/RConn1 -- K2/RConn1 -- K1/RConn1 -- V_pack_sens/LConn1
  I_shunt/RConn2 -- Battery_Pack/RConn2 -- V_pack_sens/RConn2
  R_pre/RConn1 -- K1/RConn2 -- V_bus_sens/LConn1 -- Load/RConn2 -- C_bus/LConn1
  V_dock_sens/RConn2 -- Solver/RConn1 -- V_bus_sens/RConn2 -- Charger/RConn2 -- R_dock_bleed/RConn1 -- Load/LConn1 -- C_bus/RConn1 -- GND/LConn1 -- I_shunt/LConn1
  V_dock_sens/LConn1 -- K4/RConn2 -- Charger/LConn1 -- R_dock_bleed/LConn1
  Charger_PS/RConn1 -- Charger/RConn1
  I_shunt_out/LConn1 -- I_shunt/RConn1
  K1_coil_PS/RConn1 -- K1/LConn1
  K2_coil_PS/RConn1 -- K2/LConn1
  K2/RConn2 -- R_pre/LConn1
  K4_coil_PS/RConn1 -- K4/LConn1
  Load_PS/RConn1 -- Load/RConn1
  V_bus_sens_out/LConn1 -- V_bus_sens/RConn1
  V_dock_sens_out/LConn1 -- V_dock_sens/RConn1
  V_pack_sens_out/LConn1 -- V_pack_sens/RConn1

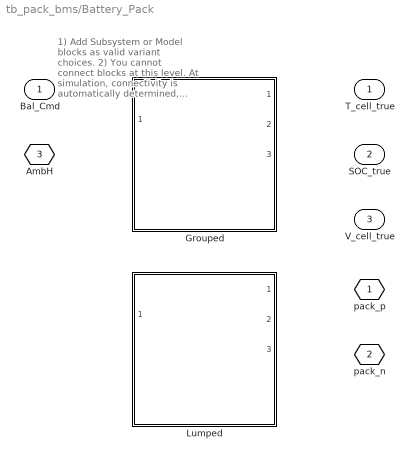
== system tb_pack_bms/Battery_Pack ==
  note: 1) Add Subsystem or Model blocks as valid variant choices.
      | 2) You cannot connect blocks at this level. At simulation, connectivity is automatically
      | determined, based on the active variant and port name matching.
  Bal_Cmd : Inport
  Grouped : Subsystem  VariantControl=VC_PACK == 1  ReferencedSubsystem=Pack_Grouped
  Lumped : Subsystem  VariantControl=VC_PACK == 2  ReferencedSubsystem=Pack_Lumped
  pack_p : PMIOPort  Side=Right  ConnectionType=Connection: foundation.electrical.electrical
  pack_n : PMIOPort  Port=2  Side=Right  ConnectionType=Connection: foundation.electrical.electrical
  AmbH : PMIOPort  Port=3  Side=Left  ConnectionType=Connection: foundation.thermal.thermal
  T_cell_true : Outport
  SOC_true : Outport  Port=2
  V_cell_true : Outport  Port=3
